simulink model "Boost_converter_hysteresis"  (R2025b)
settings: Solver=VariableStepAuto  StartTime=0.0  StopTime=1  MaxStep=1e-5  RelTol=1e-3
libraries: spsSeriesRLCBranchLib x3, spsDCVoltageSourceLib x1, spsDiodeLib x1, spsIGBTDiodeLib x1, spsVoltageMeasurementLib x1, sps_lib x1
settings Model: Creator=hp  LastModifiedBy=arif
settings OptimizationCC: ReuseModelBlockBuffer=off
settings RTWCC: GPUComputeCapability=3.5

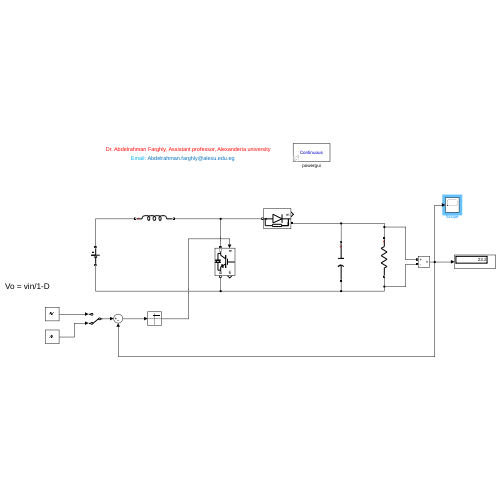
[thumbnail: Simulink's stored preview of the top-level diagram]
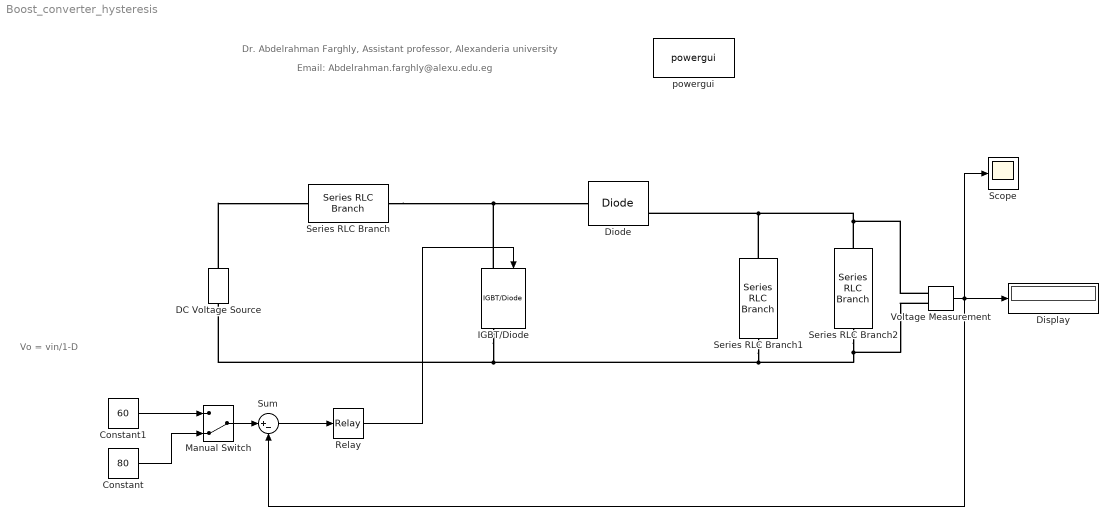
== system Boost_converter_hysteresis ==
  note: Vo = vin/1-D
  note: Email: Abdelrahman.farghly@alexu.edu.eg
  note: Dr. Abdelrahman Farghly, Assistant professor, Alexanderia university
  Constant : Constant  Value=80
  Constant1 : Constant  Value=60
  DC Voltage Source : spsDCVoltageSourceLib/DC Voltage Source  Amplitude=24  Measurements=None
  Diode : spsDiodeLib/Diode  Ron=0.001  Lon=0  Vf=0.8  IC=0  UseSnubber=0  Rs=500  Cs=250e-9  Measurements=on
  Display : Display
  IGBT/Diode : spsIGBTDiodeLib/IGBT//Diode  Ron=1e-3  Rs=1e5  Cs=inf  Measurements=on
  Manual Switch : ManualSwitch  CurrentSetting=0
  Relay : Relay  OnSwitchValue=.001  OffSwitchValue=-.001  OnOutputValue=0  OffOutputValue=1
  Scope : Scope
      settings: ActiveDisplayYMinimum=-5.0317788957050507  ActiveDisplayYMaximum=45.286010061345465
  Series RLC Branch : spsSeriesRLCBranchLib/Series RLC Branch  LConnTagsString=__new0  RConnTagsString=__new0  BranchType=L  Resistance=1  Inductance=5e-3  SetiL0=off  InitialCurrent=0  Capacitance=1e-6  Setx0=off  InitialVoltage=0  Measurements=None
  Series RLC Branch1 : spsSeriesRLCBranchLib/Series RLC Branch  LConnTagsString=__new0  RConnTagsString=__new0  BranchType=C  Resistance=1  Inductance=1e-3  SetiL0=off  InitialCurrent=0  Capacitance=330e-6  Setx0=off  InitialVoltage=0  Measurements=None
  Series RLC Branch2 : spsSeriesRLCBranchLib/Series RLC Branch  LConnTagsString=__new0  RConnTagsString=__new0  BranchType=R  Resistance=20  Inductance=1e-3  SetiL0=off  InitialCurrent=0  Capacitance=100e-6  Setx0=off  InitialVoltage=0  Measurements=None
  Sum : Sum  Inputs=|+-
  Voltage Measurement : spsVoltageMeasurementLib/Voltage Measurement  PhasorSimulation=off  OutputType=Complex  PSBequivalent=0
  powergui : sps_lib/powergui  Priority=1  SimulationMode=Continuous  SampleTime=1e-6  frequency=60  Iterations=50  frequencyindice=0  Pbase=100e6  ErrMax=1e-4  UnitsV=kV  UnitsW=MW  buscounter=0  FunctionMessages=off  echomessages=off  EnableUseOfTLC=off  CurrentSourceSwitches=off  DisableSnubberDevices=off  DisableRonSwitches=off  DisableVfSwitches=off  DisplayEquations=off  AutomaticDiscreteSolvers=off  SolverType=Tustin/Backward Euler (TBE)  Interpol=off  ExternalGateDelay=off  methode=off  Ts=100  x0status=blocks  SPID=on  SwTol=0  HookPort=off  NonlinearTolerance=1e-4  nMaxIteration=100  ContinueOnMaxIteration=off  RestoreLinks=warning  ResistiveCurrentMeasurement=off  Frange=[0:2:500]  Ylog=off  Xlog=on  ShowGrid=off  save=off  variable=ZData  structure=0  ZoomFFT=off  StartTime=0.0  cycles=1  DisplayStyle=1  fundamental=60  FreqAxis=off  MaxFrequency=1000  frequencyindicesteady=1  RmsSteady=1  display=off
  wires:
  Voltage Measurement/1 -> Scope/1, Display/1, Sum/2
  Constant1/1 -> Manual Switch/1
  Sum/1 -> Relay/1
  Relay/1 -> IGBT/Diode/1
  Manual Switch/1 -> Sum/1
  Constant/1 -> Manual Switch/2
  connections:
  Series RLC Branch2/LConn1 -- Voltage Measurement/LConn1 -- Series RLC Branch1/LConn1 -- Diode/RConn1
  DC Voltage Source/RConn1 -- Series RLC Branch/LConn1
  Series RLC Branch/RConn1 -- IGBT/Diode/LConn1 -- Diode/LConn1
  Series RLC Branch2/RConn1 -- Series RLC Branch1/RConn1 -- IGBT/Diode/RConn1 -- DC Voltage Source/LConn1 -- Voltage Measurement/LConn2
